simulink model "MSD_MSR-Rotational_Systems"  (R2025b)
settings: Solver=VariableStepAuto  StartTime=0.0  StopTime=1  RelTol=1e-9
undefined symbols (not defined in the file): gamma, k, m
libraries: fl_lib x22, nesl_utility x10, ee_lib x1
settings Model: Creator=franc  LastModifiedBy=franc

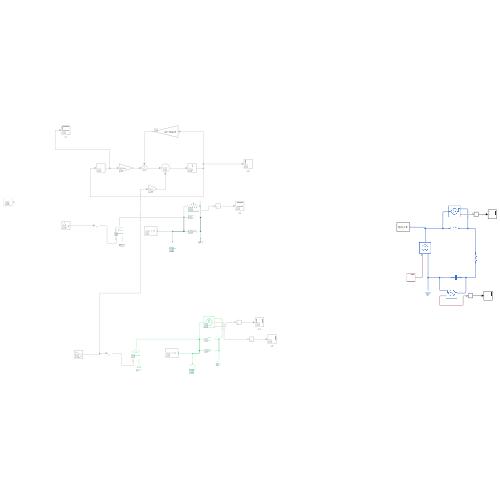
[thumbnail: Simulink's stored preview of the top-level diagram]
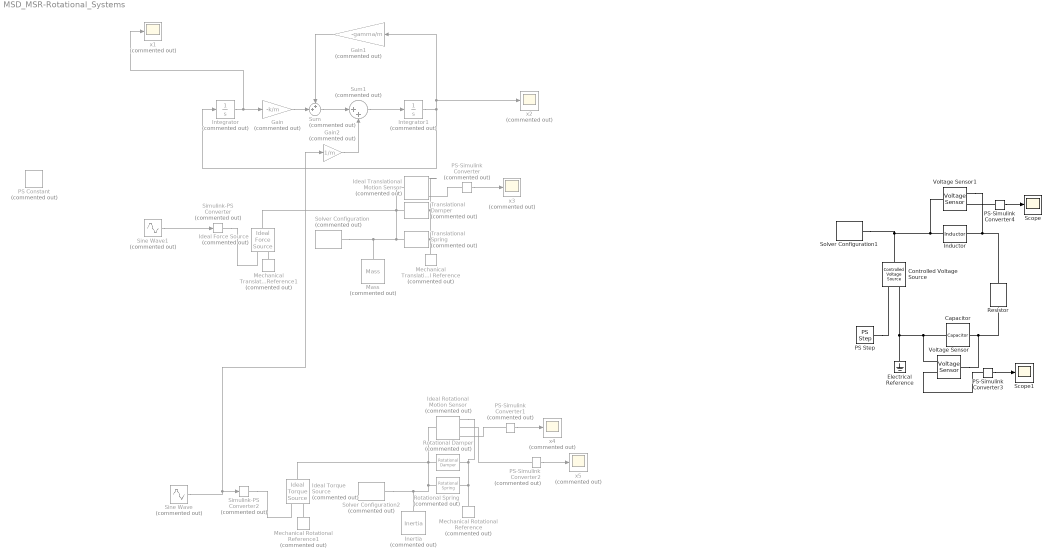
== system MSD_MSR-Rotational_Systems ==
  Capacitor : fl_lib/Electrical/Electrical Elements/Capacitor  c=1e-6 F  r=1e-6 Ohm  g=0 1/Ohm  i_specify=off  i_priority=None  i=0 A  i_nominal_specify=off  i_nominal_value=1  i_nominal_unit=A  v_specify=off  v_priority=None  v=0 V  v_nominal_specify=off  v_nominal_value=1  v_nominal_unit=V  vc_specify=off  vc_priority=High  vc=0 V  vc_nominal_specify=off  vc_nominal_value=1  vc_nominal_unit=V
  Controlled Voltage Source : fl_lib/Electrical/Electrical Sources/Controlled Voltage Source
  Electrical Reference : fl_lib/Electrical/Electrical Elements/Electrical Reference
  Gain : Gain  Commented=on  Gain=-k/m
  Gain1 : Gain  Commented=on  Gain=-gamma/m
  Gain2 : Gain  Commented=on  Gain=1/m
  Ideal Force Source : fl_lib/Mechanical/Mechanical Sources/Ideal Force Source  Commented=on
  Ideal Rotational Motion Sensor : fl_lib/Mechanical/Mechanical Sensors/Ideal Rotational Motion Sensor  Commented=on  reference=foundation.enum.MeasurementReference.difference  acceleration_port=false  velocity_port=true  position_port=true  wrap_angle=false  offset=0 rad
  Ideal Torque Source : fl_lib/Mechanical/Mechanical Sources/Ideal Torque Source  Commented=on
  Ideal Translational Motion Sensor : fl_lib/Mechanical/Mechanical Sensors/Ideal Translational Motion Sensor  Commented=on  reference=foundation.enum.MeasurementReference.difference  acceleration_port=false  velocity_port=true  position_port=true  offset=0 m
  Inductor : ee_lib/Passive/Inductor  l=1e-6 H  enable_L_tol=ee.enum.toleranceApplication.none  L_tol=20  tol_distribution=ee.enum.toleranceDistribution.uniform  nSigma=4  r=0 Ohm  g=1e-9 1/Ohm  enable_operating_limits=ee.enum.enable.no  operating_limit_action=ee.enum.passive.reportOpLim.warn  max_working_current=1 A  power_rating=1 W  i_L_specify=off  i_L_priority=High  i_L=0 A  i_L_nominal_specify=off  i_L_nominal_value=1  i_L_nominal_unit=A
  Inertia : fl_lib/Mechanical/Rotational Elements/Inertia  Commented=on  inertia=100 kg*m^2  num_ports=foundation.enum.numPorts2.one  w_specify=off  w_priority=High  w=0 rad/s  w_nominal_specify=off  w_nominal_value=1  w_nominal_unit=rad/s  t_specify=off  t_priority=None  t=0 N*m  t_nominal_specify=off  t_nominal_value=1  t_nominal_unit=N*m
  Integrator : Integrator  Commented=on
  Integrator1 : Integrator  Commented=on
  Mass : fl_lib/Mechanical/Translational Elements/Mass  Commented=on  mass=10 kg  num_ports=foundation.enum.numPorts2.one  v_specify=off  v_priority=High  v=0 m/s  v_nominal_specify=off  v_nominal_value=1  v_nominal_unit=m/s  f_specify=off  f_priority=None  f=0 N  f_nominal_specify=off  f_nominal_value=1  f_nominal_unit=N
  Mechanical Rotational Reference : fl_lib/Mechanical/Rotational Elements/Mechanical Rotational Reference  Commented=on
  Mechanical Rotational Reference1 : fl_lib/Mechanical/Rotational Elements/Mechanical Rotational Reference  Commented=on
  Mechanical Translational Reference : fl_lib/Mechanical/Translational Elements/Mechanical Translational Reference  Commented=on
  Mechanical Translational Reference1 : fl_lib/Mechanical/Translational Elements/Mechanical Translational Reference  Commented=on
  PS Constant : fl_lib/Physical Signals/Sources/PS Constant  Commented=on  constant=1
  PS Step : fl_lib/Physical Signals/Sources/PS Step  step_time=0 s  initial_value=0  final_value=20
  PS-Simulink Converter : nesl_utility/PS-Simulink Converter  Commented=on  PhysicalDomain=network_engine_domain  SubClassName=ps_output  LeftPortType=input  RightPortType=output  PseudoPeriodic=off  Frequencies=[]  VectorFormat=inherit  Unit=m  AffineConversion=off
  PS-Simulink Converter1 : nesl_utility/PS-Simulink Converter  Commented=on  PhysicalDomain=network_engine_domain  SubClassName=ps_output  LeftPortType=input  RightPortType=output  PseudoPeriodic=off  Frequencies=[]  VectorFormat=inherit  Unit=rad  AffineConversion=off
  PS-Simulink Converter2 : nesl_utility/PS-Simulink Converter  Commented=on  PhysicalDomain=network_engine_domain  SubClassName=ps_output  LeftPortType=input  RightPortType=output  PseudoPeriodic=off  Frequencies=[]  VectorFormat=inherit  Unit=rad/s  AffineConversion=off
  PS-Simulink Converter3 : nesl_utility/PS-Simulink Converter  PhysicalDomain=network_engine_domain  SubClassName=ps_output  LeftPortType=input  RightPortType=output  PseudoPeriodic=off  Frequencies=[]  VectorFormat=inherit  Unit=inherit  AffineConversion=off
  PS-Simulink Converter4 : nesl_utility/PS-Simulink Converter  PhysicalDomain=network_engine_domain  SubClassName=ps_output  LeftPortType=input  RightPortType=output  PseudoPeriodic=off  Frequencies=[]  VectorFormat=inherit  Unit=inherit  AffineConversion=off
  Resistor : fl_lib/Electrical/Electrical Elements/Resistor  R=1 Ohm  i_specify=off  i_priority=None  i=0 A  i_nominal_specify=off  i_nominal_value=1  i_nominal_unit=A  v_specify=off  v_priority=None  v=0 V  v_nominal_specify=off  v_nominal_value=1  v_nominal_unit=V
  Rotational Damper : fl_lib/Mechanical/Rotational Elements/Rotational Damper  Commented=on  D=7841.4 N*m*s/rad  w_specify=off  w_priority=None  w=0 rad/s  w_nominal_specify=off  w_nominal_value=1  w_nominal_unit=rad/s  t_specify=off  t_priority=None  t=0 N*m  t_nominal_specify=off  t_nominal_value=1  t_nominal_unit=N*m
  Rotational Spring : fl_lib/Mechanical/Rotational Elements/Rotational Spring  Commented=on  spr_rate=313600 N*m/rad  w_specify=off  w_priority=None  w=0 rad/s  w_nominal_specify=off  w_nominal_value=1  w_nominal_unit=rad/s  t_specify=off  t_priority=None  t=0 N*m  t_nominal_specify=off  t_nominal_value=1  t_nominal_unit=N*m  phi_specify=off  phi_priority=High  phi=0 rad  phi_nominal_specify=off  phi_nominal_value=1  phi_nominal_unit=rad
  Scope : Scope
      settings: ActiveDisplayYMinimum=-0.46055330876162981  ActiveDisplayYMaximum=1.1622836998624024  DataLoggingVariableName=ScopeData5
  Scope1 : Scope
      settings: ActiveDisplayYMinimum=-0.14537828577505371  ActiveDisplayYMaximum=1.3084045719754938  DataLoggingVariableName=ScopeData6
  Simulink-PS Converter : nesl_utility/Simulink-PS Converter  Commented=on  PhysicalDomain=network_engine_domain  SubClassName=ps_input  LeftPortType=input  RightPortType=output  PseudoPeriodic=off  Frequencies=[]  NoiseDistribution=none  NoiseParameters=[]  Unit=N  AffineConversion=off  FilteringAndDerivatives=provide  SimscapeFilterOrder=1  InputFilterTimeConstant=0.001  UdotUserProvided=0
  Simulink-PS Converter2 : nesl_utility/Simulink-PS Converter  Commented=on  PhysicalDomain=network_engine_domain  SubClassName=ps_input  LeftPortType=input  RightPortType=output  PseudoPeriodic=off  Frequencies=[]  NoiseDistribution=none  NoiseParameters=[]  Unit=N*m  AffineConversion=off  FilteringAndDerivatives=provide  SimscapeFilterOrder=1  InputFilterTimeConstant=0.001  UdotUserProvided=0
  Sine Wave : Sin  Commented=on  Amplitude=313600  SampleTime=0
  Sine Wave1 : Sin  Commented=on  Amplitude=1/1960  SampleTime=0
  Solver Configuration : nesl_utility/Solver Configuration  Commented=on  PhysicalDomain=network_engine_domain  SubClassName=solver  LeftPortType=input  RightPortType=generic  Tones=[]  Harmonics=[]  SimulateNoise=off  Profile=off  UseLocalSampling=off  EnableSwitchedLinearOptims=on  FrequencyDomain=off  UseCCode=off  RelTol=0.001  AbsTol=0.001  MinStep=1e-09  ToWorkspace=off  RevertToSquareIcSolve=off  NumHomotopyIterations=100  PhasorMode=off  PhasorModeNumHarmonics=1  ConsistencySolver=NEWTON_XTOL_AFTER_FTOL  IndexReductionMethod=DerivativeReplacement  DoDC=off  ResidualTolerance=1e-09  ConsistencyTolSource=GLOBAL  ConsistencyAbsTol=0.001  ConsistencyRelTol=0.001  ConsistencyTolFactor=0.001  UseLocalSolver=off  LocalSolverChoice=NE_BACKWARD_EULER_ADVANCER  ResolveIndetEquations=on  FunctionEvalNumThread=1  LocalSolverSampleTime=0.001  DoFixedCost=off  MaxNonlinIter=3  MaxModeIter=2  ComputeImpulses=off  ImpulseIterations=2  LinearAlgebra=auto  LinearAlgebraNumThread=0  EquationFormulation=NE_TIME_EF  DelaysMemoryBudget=1024  AutomaticFiltering=on  FilteringTimeConstant=0.001  PartitionStorageMethod=AS_NEEDED  PartitionMemoryBudget=1024  PartitionMethod=ROBUST  MultibodyUseLocalSolver=off  MultibodyLocalSolverChoice=ODE1  MultibodyLocalSolverSampleTime=0.001
  Solver Configuration1 : nesl_utility/Solver Configuration  PhysicalDomain=network_engine_domain  SubClassName=solver  LeftPortType=input  RightPortType=generic  Tones=[]  Harmonics=[]  SimulateNoise=off  Profile=off  UseLocalSampling=off  EnableSwitchedLinearOptims=on  FrequencyDomain=off  UseCCode=off  RelTol=0.001  AbsTol=0.001  MinStep=1e-09  ToWorkspace=off  RevertToSquareIcSolve=off  NumHomotopyIterations=100  PhasorMode=off  PhasorModeNumHarmonics=1  ConsistencySolver=NEWTON_XTOL_AFTER_FTOL  IndexReductionMethod=DerivativeReplacement  DoDC=off  ResidualTolerance=1e-09  ConsistencyTolSource=GLOBAL  ConsistencyAbsTol=0.001  ConsistencyRelTol=0.001  ConsistencyTolFactor=0.001  UseLocalSolver=off  LocalSolverChoice=NE_BACKWARD_EULER_ADVANCER  ResolveIndetEquations=on  FunctionEvalNumThread=1  LocalSolverSampleTime=0.001  DoFixedCost=off  MaxNonlinIter=3  MaxModeIter=2  ComputeImpulses=off  ImpulseIterations=2  LinearAlgebra=auto  LinearAlgebraNumThread=0  EquationFormulation=NE_TIME_EF  DelaysMemoryBudget=1024  AutomaticFiltering=on  FilteringTimeConstant=0.001  PartitionStorageMethod=AS_NEEDED  PartitionMemoryBudget=1024  PartitionMethod=ROBUST  MultibodyUseLocalSolver=off  MultibodyLocalSolverChoice=ODE1  MultibodyLocalSolverSampleTime=0.001
  Solver Configuration2 : nesl_utility/Solver Configuration  Commented=on  PhysicalDomain=network_engine_domain  SubClassName=solver  LeftPortType=input  RightPortType=generic  Tones=[]  Harmonics=[]  SimulateNoise=off  Profile=off  UseLocalSampling=off  EnableSwitchedLinearOptims=on  FrequencyDomain=off  UseCCode=off  RelTol=0.001  AbsTol=0.001  MinStep=1e-09  ToWorkspace=off  RevertToSquareIcSolve=off  NumHomotopyIterations=100  PhasorMode=off  PhasorModeNumHarmonics=1  ConsistencySolver=NEWTON_XTOL_AFTER_FTOL  IndexReductionMethod=DerivativeReplacement  DoDC=off  ResidualTolerance=1e-09  ConsistencyTolSource=GLOBAL  ConsistencyAbsTol=0.001  ConsistencyRelTol=0.001  ConsistencyTolFactor=0.001  UseLocalSolver=off  LocalSolverChoice=NE_BACKWARD_EULER_ADVANCER  ResolveIndetEquations=on  FunctionEvalNumThread=1  LocalSolverSampleTime=0.001  DoFixedCost=off  MaxNonlinIter=3  MaxModeIter=2  ComputeImpulses=off  ImpulseIterations=2  LinearAlgebra=auto  LinearAlgebraNumThread=0  EquationFormulation=NE_TIME_EF  DelaysMemoryBudget=1024  AutomaticFiltering=on  FilteringTimeConstant=0.001  PartitionStorageMethod=AS_NEEDED  PartitionMemoryBudget=1024  PartitionMethod=ROBUST  MultibodyUseLocalSolver=off  MultibodyLocalSolverChoice=ODE1  MultibodyLocalSolverSampleTime=0.001
  Sum : Sum  Commented=on  Inputs=++|
  Sum1 : Sum  Commented=on  Inputs=|++
  Translational Damper : fl_lib/Mechanical/Translational Elements/Translational Damper  Commented=on  D=196 N*s/m  v_specify=off  v_priority=None  v=0 m/s  v_nominal_specify=off  v_nominal_value=1  v_nominal_unit=m/s  f_specify=off  f_priority=None  f=0 N  f_nominal_specify=off  f_nominal_value=1  f_nominal_unit=N
  Translational Spring : fl_lib/Mechanical/Translational Elements/Translational Spring  Commented=on  spr_rate=1960 N/m  v_specify=off  v_priority=None  v=0 m/s  v_nominal_specify=off  v_nominal_value=1  v_nominal_unit=m/s  f_specify=off  f_priority=None  f=0 N  f_nominal_specify=off  f_nominal_value=1  f_nominal_unit=N  x_specify=off  x_priority=High  x=0 m  x_nominal_specify=off  x_nominal_value=1  x_nominal_unit=m
  Voltage Sensor : fl_lib/Electrical/Electrical Sensors/Voltage Sensor
  Voltage Sensor1 : fl_lib/Electrical/Electrical Sensors/Voltage Sensor
  x{1..5} (5 alike) : Scope  Commented=on
      x1 settings: ActiveDisplayYMinimum=-1  ActiveDisplayYMaximum=1
      x2 settings: ActiveDisplayYMinimum=-0.48327682689354862  ActiveDisplayYMaximum=0.45082095630209362
      x3 settings: ActiveDisplayYMinimum=-3.2541423127046455E-7  ActiveDisplayYMaximum=3.2541422967127736E-7  DataLoggingVariableName=ScopeData2
      x4 settings: ActiveDisplayYMinimum=-0.12500071843399535  ActiveDisplayYMaximum=1.1250064659059584  DataLoggingVariableName=ScopeData3
      x5 settings: ActiveDisplayYMinimum=-4.5339555933351932  ActiveDisplayYMaximum=29.025369368450537  DataLoggingVariableName=ScopeData4
  wires:
  Integrator/1 -> x1/1, Gain/1
  Gain/1 -> Sum/2
  Gain1/1 -> Sum/1
  Sum/1 -> Sum1/1
  Sum1/1 -> Integrator1/1
  Integrator1/1 -> Gain1/1, x2/1, Integrator/1
  Gain2/1 -> Sum1/2
  Sine Wave1/1 -> Simulink-PS Converter/1
  PS-Simulink Converter/1 -> x3/1
  PS-Simulink Converter1/1 -> x4/1
  Sine Wave/1 -> Gain2/1, Simulink-PS Converter2/1
  PS-Simulink Converter2/1 -> x5/1
  PS-Simulink Converter4/1 -> Scope/1
  PS-Simulink Converter3/1 -> Scope1/1
  connections:
  Mechanical Translational Reference/LConn1 -- Ideal Translational Motion Sensor/RConn1 -- Translational Damper/RConn1 -- Translational Spring/RConn1
  Mass/LConn1 -- Solver Configuration/RConn1 -- Translational Damper/LConn1 -- Ideal Translational Motion Sensor/LConn1 -- Ideal Force Source/LConn1 -- Translational Spring/LConn1
  Mechanical Translational Reference1/LConn1 -- Ideal Force Source/RConn2
  Simulink-PS Converter/RConn1 -- Ideal Force Source/RConn1
  PS-Simulink Converter/LConn1 -- Ideal Translational Motion Sensor/RConn3
  Rotational Damper/LConn1 -- Ideal Torque Source/LConn1 -- Ideal Rotational Motion Sensor/LConn1 -- Inertia/LConn1 -- Solver Configuration2/RConn1 -- Rotational Spring/LConn1
  Rotational Damper/RConn1 -- Ideal Rotational Motion Sensor/RConn1 -- Mechanical Rotational Reference/LConn1 -- Rotational Spring/RConn1
  PS-Simulink Converter1/LConn1 -- Ideal Rotational Motion Sensor/RConn3
  Simulink-PS Converter2/RConn1 -- Ideal Torque Source/RConn1
  Mechanical Rotational Reference1/LConn1 -- Ideal Torque Source/RConn2
  PS-Simulink Converter2/LConn1 -- Ideal Rotational Motion Sensor/RConn2
  Capacitor/RConn1 -- Voltage Sensor/RConn2 -- Electrical Reference/LConn1 -- Controlled Voltage Source/RConn2
  Inductor/LConn1 -- Voltage Sensor1/LConn1 -- Solver Configuration1/RConn1 -- Controlled Voltage Source/LConn1
  Resistor/LConn1 -- Voltage Sensor1/RConn2 -- Inductor/RConn1
  Capacitor/LConn1 -- Voltage Sensor/LConn1 -- Resistor/RConn1
  PS Step/RConn1 -- Controlled Voltage Source/RConn1
  PS-Simulink Converter4/LConn1 -- Voltage Sensor1/RConn1
  Voltage Sensor/RConn1 -- PS-Simulink Converter3/LConn1
